simulink model "quartercar_PID_Passive"  (R2023a)
settings: Solver=VariableStepAuto  StartTime=0  StopTime=10  FixedStep=0.05  RelTol=1e-5  EnableMultiTasking=on
model workspace (MAT data in the model file):
  cs = 2126
  ks = 24000
  kt = 243000
  ms = 365
  mu = 43
libraries: simulink x2, slpidlib x1
settings Model: Creator=Administrator  LastModifiedBy=Yuk
settings SolverCC: AllowMultiTaskInputOutput=on  InsertRTBMode=Never (minimum delay)
settings DataIOCC: SaveFormat=Array
settings OptimizationCC: LifeSpan=inf
settings DebuggingCC: AlgebraicLoopMsg=none  UnderspecifiedInitializationDetection=Classic  MergeDetectMultiDrivingBlocksExec=none  SolverPrmCheckMsg=warning  UnconnectedInputMsg=warning  UnconnectedOutputMsg=warning  UnconnectedLineMsg=warning  StateNameClashWarn=warning  SFUnexpectedBacktrackingDiag=warning  SFNoUnconditionalDefaultTransitionDiag=warning  SFExecutionAtInitializationDiag=none  ArithmeticOperatorsInVariantConditions=warning
settings HardwareCC: ProdBitPerPointer=32  ProdBitPerSizeT=32  ProdBitPerPtrDiffT=32  ProdLargestAtomicFloat=None  ProdIntDivRoundTo=Undefined  ProdEndianess=Unspecified  ProdWordSize=32  ProdHWDeviceType=32-bit Generic
settings ModelReferenceCC: PropagateSignalLabelsOutOfModel=off
settings SFSimCC: SimUseLocalCustomCode=off  CustomCodeUndefinedFunction=UseInterfaceOnly  SimTargetLang=C++
settings RTWCC: RTWUseLocalCustomCode=off
settings CodeAppCC: StateflowObjectComments=on
settings GRTTargetCC: TargetLangStandard=C89/C90 (ANSI)
settings ConfigComp: CovMetricSettings=dw  CovSaveCumulativeToWorkspaceVar=on  CovSaveSingleToWorkspaceVar=on  CovExternalEMLEnable=off

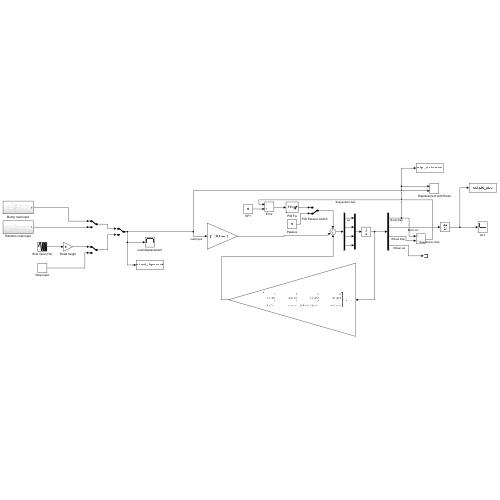
[thumbnail: Simulink's stored preview of the top-level diagram]
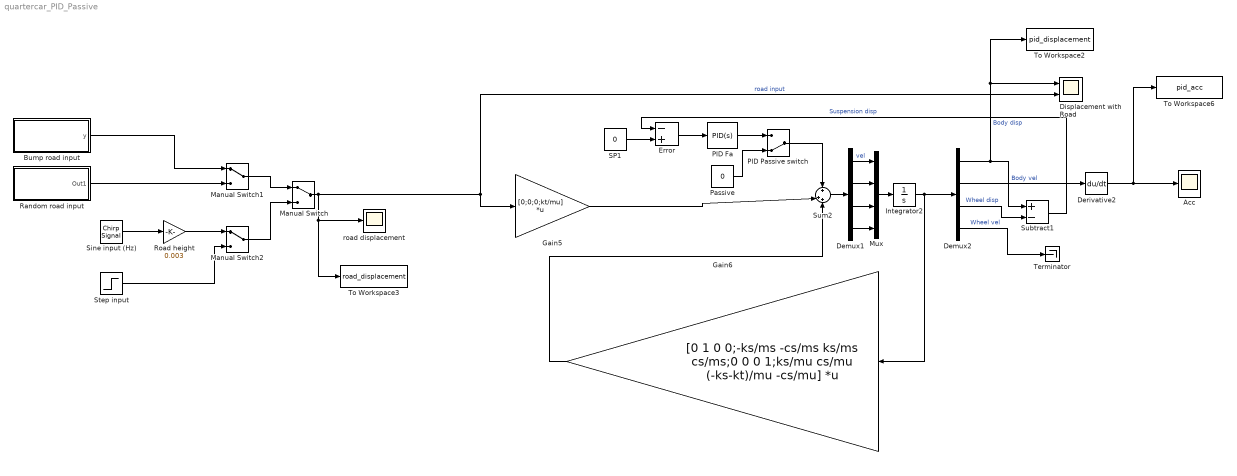
== system quartercar_PID_Passive ==
  Acc : Scope
  Bump road input : Subsystem
  Demux1 : Demux
  Demux2 : Demux
  Derivative2 : Derivative
  Displacement with Road : Scope  NumInputPorts=2
  Error : Sum  Inputs=-+
  Gain5 : Gain  Gain=[0;0;0;kt/mu]  Multiplication=Matrix(K*u)
  Gain6 : Gain  Gain=[0 1 0 0;-ks/ms -cs/ms ks/ms cs/ms;0 0 0 1;ks/mu cs/mu (-ks-kt)/mu -cs/mu]  Multiplication=Matrix(K*u)
  Integrator2 : Integrator
  Manual Switch : ManualSwitch
  Manual Switch1 : ManualSwitch
  Manual Switch2 : ManualSwitch
  Mux : Mux
  PID Fa : slpidlib/PID Controller  Controller=PID  Form=Parallel  TimeDomain=Continuous-time  UseExternalTs=off  SampleTime=1  IntegratorMethod=Forward Euler  FilterMethod=Forward Euler  ControllerParametersSource=internal  P=0.8  I=0.1  UseKiTs=off  D=0.5  N=100  UseFilter=on  TunerSelectOption=Transfer Function Based (PID Tuner App)  InitialConditionSource=internal  InitialConditionForIntegrator=0  InitialConditionForFilter=0  DifferentiatorICPrevScaledInput=0  ExternalReset=none  TrackingMode=off  Kt=1  LimitOutput=on  SatLimitsSource=internal  UpperSaturationLimit=4000  LowerSaturationLimit=-4000  LinearizeAsGain=off  AntiWindupMode=none  Kb=1  LimitIntegrator=off  UpperIntegratorSaturationLimit=inf  LowerIntegratorSaturationLimit=-inf  POutMin=[]  POutMax=[]  IOutMin=[]  IOutMax=[]  DOutMin=[]  DOutMax=[]  NOutMin=[]  NOutMax=[]  SumOutMin=[]  SumOutMax=[]  SaturationOutMin=[]  SaturationOutMax=[]  PParamMin=[]  PParamMax=[]  IParamMin=[]  IParamMax=[]  DParamMin=[]  DParamMax=[]  NParamMin=[]  NParamMax=[]  KbParamMin=[]  KbParamMax=[]  KtParamMin=[]  KtParamMax=[]  KbOutMin=[]  KbOutMax=[]  KtOutMin=[]  KtOutMax=[]  IntegratorOutMin=[]  IntegratorOutMax=[]  FilterOutMin=[]  FilterOutMax=[]  SumI1OutMin=[]  SumI1OutMax=[]  SumI2OutMin=[]  SumI2OutMax=[]  SumI3OutMin=[]  SumI3OutMax=[]  SumI4OutMin=[]  SumI4OutMax=[]  SumDOutMin=[]  SumDOutMax=[]  DifferentiatorOutMin=[]  DifferentiatorOutMax=[]  FilterDiffOutCoefMin=[]  FilterDiffOutCoefMax=[]  ReciprocalOutMin=[]  ReciprocalOutMax=[]  SumDenOutMin=[]  SumDenOutMax=[]  SumNumOutMin=[]  SumNumOutMax=[]  DivideOutMin=[]  DivideOutMax=[]  UdiffTsProdOutMin=[]  UdiffTsProdOutMax=[]  NTsProdOutMin=[]  NTsProdOutMax=[]  UintegralTsProdOutMin=[]  UintegralTsProdOutMax=[]  UngainTsProdOutMin=[]  UngainTsProdOutMax=[]  ClampingZeroOutDataTypeStr=Inherit: Inherit via back propagation  ClampingZeroOutMin=[]  ClampingZeroOutMax=[]  FilterDenConstantOutDataTypeStr=Inherit: Inherit via back propagation  FilterDenConstantOutMin=[]  FilterDenConstantOutMax=[]  PCopyOutDataTypeStr=Inherit: Inherit via back propagation  PCopyOutMin=[]  PCopyOutMax=[]  NCopyOutDataTypeStr=Inherit: Inherit via back propagation  NCopyOutMin=[]  NCopyOutMax=[]  IntegratorContinuousStateAttributes=''  IntegratorStateMustResolveToSignalObject=off  IntegratorRTWStateStorageClass=Auto  FilterContinuousStateAttributes=''  FilterStateMustResolveToSignalObject=off  FilterRTWStateStorageClass=Auto  ParallelPVariant=InternalParameters  IdealPVariant=Disabled  IVariant=InternalParameters  DVariant=InternalParameters  IntegratorVariant=Continuous  SatVariant=Enabled  AWVariant=Passthrough  PCopyVariant=Disabled  TRVariant=Disabled  FdbkBlocksVariant=Forward  IdealPFdbkVariant=Disabled  SatFdbkVariant=Disabled  DerivativeFilterVariant=ContFilter  NVariant=InternalParameters  NCopyVariant=Disabled  FilterICVariant=InternalICsFilter  IntegratorICVariant=InternalICs  ExternalResetVariant=Disabled  TRSumVariant=Passthrough  SumFdbkVariant=Disabled  SumVariant=Sum_PID  TsampFilterVariant=InternalTs  TsampNgainVariant=Passthrough  TsampIntegralVariant=Disabled_SignalSpec  ExternalSaturationOutDataTypeStr=Inherit: Same as second input
  PID Passive switch : ManualSwitch  CurrentSetting=0
  Passive : Constant  Value=0
  Random road input : Subsystem
  Road height : Gain  Gain=0.003
  SP1 : Constant  Value=0
  Sine input (Hz) : simulink/Sources/Chirp Signal  f1=1  T=10  f2=1
  Step input : Step  SampleTime=0
  Subtract1 : Sum  Inputs=+-
  Sum2 : Sum  Inputs=+|++
  Terminator : Terminator
  To Workspace2 : ToWorkspace  VariableName=pid_displacement  SaveFormat=Timeseries  SampleTime=-1
  To Workspace3 : ToWorkspace  VariableName=road_displacement  SaveFormat=Timeseries  SampleTime=-1
  To Workspace6 : ToWorkspace  VariableName=pid_acc  SaveFormat=Timeseries  SampleTime=0.05
  road displacement : Scope
  wires:
  Manual Switch1/1 -> Manual Switch/1
  Manual Switch2/1 -> Manual Switch/2
  Gain6/1 -> Sum2/3
  Subtract1/1 -> Error/1  "Suspension disp"
  Sum2/1 -> Demux1/1
  Demux2/1 -> Displacement with Road/1, To Workspace2/1, Subtract1/1  "Body disp"
  Demux2/3 -> Subtract1/2  "Wheel disp"
  Gain5/1 -> Sum2/2
  Manual Switch/1 -> Gain5/1, Displacement with Road/2, To Workspace3/1, road displacement/1  "road input"
  SP1/1 -> Error/2
  Error/1 -> PID Fa/1
  Integrator2/1 -> Gain6/1, Demux2/1
  Demux2/2 -> Derivative2/1  "Body vel"
  Derivative2/1 -> Acc/1, To Workspace6/1
  Road height/1 -> Manual Switch2/1
  Sine input (Hz)/1 -> Road height/1
  Demux1/1 -> Mux/1  "vel"
  Demux1/2 -> Mux/2
  Demux1/3 -> Mux/3
  Demux1/4 -> Mux/4
  Mux/1 -> Integrator2/1
  PID Fa/1 -> PID Passive switch/1
  PID Passive switch/1 -> Sum2/1
  Passive/1 -> PID Passive switch/2
  Random road input/1(Out1) -> Manual Switch1/2
  Bump road input/1(y) -> Manual Switch1/1
  Step input/1 -> Manual Switch2/2
  Demux2/4 -> Terminator/1  "Wheel vel"

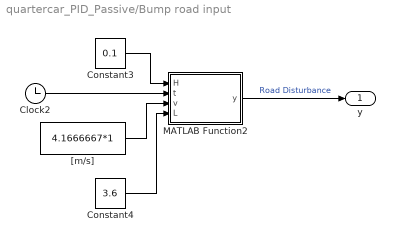
== system quartercar_PID_Passive/Bump road input ==
  Clock2 : Clock
  Constant3 : Constant  Value=0.1
  Constant4 : Constant  Value=3.6
  MATLAB Function2 : MATLAB Function  TreatAsAtomicUnit=on
  "[m/s]" : Constant  Value=4.1666667*1
  y : Outport
  wires:
  Clock2/1 -> MATLAB Function2/2(t)
  Constant4/1 -> MATLAB Function2/4(L)
  MATLAB Function2/1(y) -> y/1  "Road Disturbance"
  Constant3/1 -> MATLAB Function2/1(H)
  "[m/s]"/1 -> MATLAB Function2/3(v)

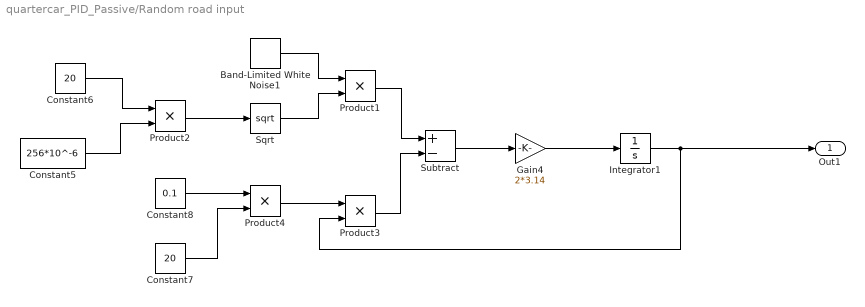
== system quartercar_PID_Passive/Random road input ==
  Band-Limited White Noise1 : simulink/Sources/Band-Limited White Noise  Cov=[5.4*10^-3]  Ts=0.1  seed=[23341]
  Constant5 : Constant  Value=256*10^-6
  Constant6 : Constant  Value=20
  Constant7 : Constant  Value=20
  Constant8 : Constant  Value=0.1
  Gain4 : Gain  Gain=2*3.14
  Integrator1 : Integrator
  Product{1..4} (4 alike) : Product
  Sqrt : Sqrt
  Subtract : Sum  Inputs=+-
  Out1 : Outport
  wires:
  Subtract/1 -> Gain4/1
  Product2/1 -> Sqrt/1
  Constant8/1 -> Product4/1
  Constant7/1 -> Product4/2
  Product4/1 -> Product3/1
  Constant6/1 -> Product2/1
  Gain4/1 -> Integrator1/1
  Integrator1/1 -> Product3/2, Out1/1
  Product1/1 -> Subtract/1
  Band-Limited White Noise1/1 -> Product1/1
  Product3/1 -> Subtract/2
  Sqrt/1 -> Product1/2
  Constant5/1 -> Product2/2

== matlab function quartercar_PID_Passive/Bump road input/MATLAB Function2 ==
  data: H input; y output; t input; v input; L input
function y = fcn(H,t,v,L)
% CODE GENERATION
if (0.5<t) && (t<L/v+0.5)
    
  y=H/2*(1-cos((2*pi*v/L)*(t-0.5)));
% w = 2*pi*v/L;
%   y=H*(1-cos(w*t));

else
    y=0;
end
out=y;
